simulink model "missile_plant_test"  (R2025a)
settings: Solver=FixedStepDiscrete  StartTime=0.0  StopTime=4  FixedStep=1/48  RelTol=1e-3
InitFcn:
  | addpath(fileparts(fileparts(get_param(bdroot,'FileName'))));addpath(fileparts(get_param(bdroot,'FileName')));
model workspace (MAT data in the model file):
  benchOptions.closedLoop = 0
  benchOptions.missile = 'su_r_77_1'
  benchOptions.duration = 4
  benchOptions.axis = 2
  benchOptions.amplitude = 1
  benchOptions.startTime = 0.5
  benchOptions.pulseWidth = 0.0208333333333
  benchOptions.signal = 'step'
  benchOptions.freeFlight = 0
  benchOptions.condition.height = 5000
  benchOptions.condition.speed = 600
  benchOptions.condition.time = 6
  benchOptions.wind = [0; 0; 0]
settings Model: Creator=skyking  LastModifiedBy=skyking

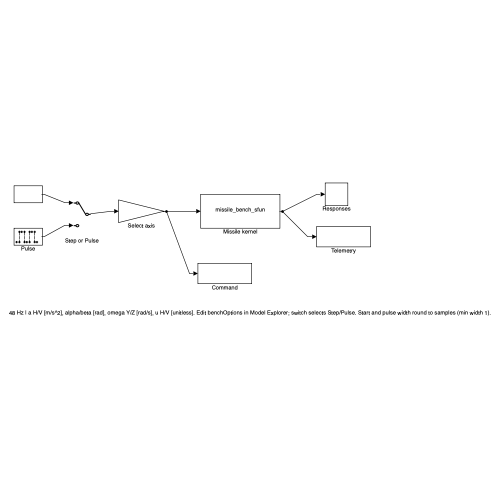
[thumbnail: Simulink's stored preview of the top-level diagram]
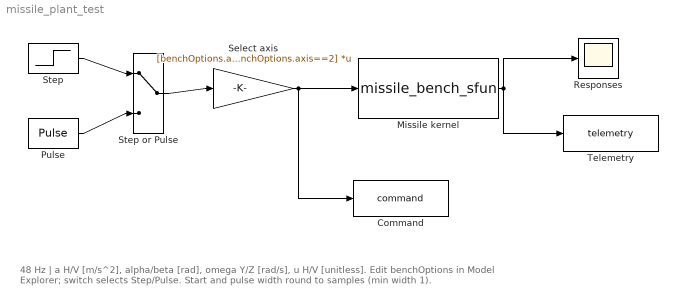
== system missile_plant_test ==
  note: 48 Hz | a H/V [m/s^2], alpha/beta [rad], omega Y/Z [rad/s], u H/V [unitless]. Edit benchOptions in Model Explorer; switch selects Step/Pulse. Start and pulse width round to samples (min width 1).
  Command : ToWorkspace  VariableName=command  SaveFormat=Timeseries  SampleTime=-1
  Missile kernel : M-S-Function  FunctionName=missile_bench_sfun  Parameters=benchOptions
  Pulse : DiscretePulseGenerator  Amplitude=benchOptions.amplitude  Period=100000  PulseWidth=max(1,round(benchOptions.pulseWidth*48))  PhaseDelay=round(benchOptions.startTime*48)  SampleTime=1/48
  Responses : Scope
  Select axis : Gain  Gain=[benchOptions.axis==1;benchOptions.axis==2]  Multiplication=Matrix(K*u)
  Step : Step  Time=round(benchOptions.startTime*48)/48  After=benchOptions.amplitude  SampleTime=1/48
  Step or Pulse : ManualSwitch
  Telemetry : ToWorkspace  VariableName=telemetry  SaveFormat=Timeseries  SampleTime=-1
  wires:
  Step/1 -> Step or Pulse/1
  Pulse/1 -> Step or Pulse/2
  Step or Pulse/1 -> Select axis/1
  Select axis/1 -> Missile kernel/1, Command/1
  Missile kernel/1 -> Responses/1, Telemetry/1
